simulink model "DPWMA_17_Level_Rectifier_Dual_PI"  (R2021b)
settings: Solver=VariableStepAuto  StartTime=0.0  StopTime=0.5  RelTol=1e-3
libraries: spsSeriesRLCBranchLib x51, spsVoltageMeasurementLib x27, spsDiodeLib x24, spsIGBTDiodeLib x24, simulink x24, spsUniversalBridgeLib x24, slpidlib x3, spsACVoltageSourceLib x3, spsCurrentMeasurementLib x2, spsMeanLib x2, spsRMSLib x2, spsTHDLib x1
(part 3 of 3)

== system DPWMA_17_Level_Rectifier_Dual_PI/Subsystem2/子模块6 ==
  M : Inport
  C : spsSeriesRLCBranchLib/Series RLC Branch  LConnTagsString=__new0  RConnTagsString=__new0  BranchType=C  Resistance=0  Inductance=0  SetiL0=off  InitialCurrent=0  Capacitance=4e-3  Setx0=on  InitialVoltage=1000  Measurements=None
  Diode : spsDiodeLib/Diode  Ron=0.001  Lon=0  Vf=2  IC=0  UseSnubber=0  Rs=1e6  Cs=2e-9  Measurements=off
  IGBT/Diode : spsIGBTDiodeLib/IGBT//Diode  Ron=1e-3  Rs=1e5  Cs=inf  Measurements=off
  R : spsSeriesRLCBranchLib/Series RLC Branch  LConnTagsString=__new0  RConnTagsString=__new0  BranchType=R  Resistance=15  Inductance=0  SetiL0=off  InitialCurrent=0  Capacitance=2e-3  Setx0=on  InitialVoltage=311  Measurements=None
  Subsystem2 : Subsystem
  Universal Bridge : spsUniversalBridgeLib/Universal Bridge  Arms=2  SnubberResistance=0.01  SnubberCapacitance=1e-8  Device=Diodes  Ron=1e-3  Lon=0  ForwardVoltages="[  0  0  ]"  ForwardVoltage=3  GTOparameters=[ 10e-6 , 20e-6 ]  IGBTparameters=[ 1e-6 , 2e-6 ]  Measurements=None  Measurements_2=None  converterType=Rectifier
  Vm1 : spsVoltageMeasurementLib/Voltage Measurement  PhasorSimulation=off  OutputType=Complex  PSBequivalent=0
  + : PMIOPort  Side=Left
  - : PMIOPort  Port=2  Side=Left
  A : PMIOPort  Port=3  Side=Right
  B : PMIOPort  Port=4  Side=Right
  Out1 : Outport
  wires:
  Subsystem2/1(g1) -> IGBT/Diode/1
  M/1 -> Subsystem2/1(MOD)
  Vm1/1 -> Out1/1
  connections:
  Diode/LConn1 -- Universal Bridge/RConn1 -- IGBT/Diode/LConn1
  B/RConn1 -- Universal Bridge/LConn2
  A/RConn1 -- Universal Bridge/LConn1
  Diode/RConn1 -- C/LConn1 -- R/LConn1 -- Vm1/LConn1
  IGBT/Diode/RConn1 -- C/RConn1 -- R/RConn1 -- Vm1/LConn2 -- Universal Bridge/RConn2

== system DPWMA_17_Level_Rectifier_Dual_PI/Subsystem2/子模块7 ==
  M : Inport
  C : spsSeriesRLCBranchLib/Series RLC Branch  LConnTagsString=__new0  RConnTagsString=__new0  BranchType=C  Resistance=0  Inductance=0  SetiL0=off  InitialCurrent=0  Capacitance=4e-3  Setx0=on  InitialVoltage=1000  Measurements=None
  Diode : spsDiodeLib/Diode  Ron=0.001  Lon=0  Vf=2  IC=0  UseSnubber=0  Rs=1e6  Cs=2e-9  Measurements=off
  IGBT/Diode : spsIGBTDiodeLib/IGBT//Diode  Ron=1e-3  Rs=1e5  Cs=inf  Measurements=off
  R : spsSeriesRLCBranchLib/Series RLC Branch  LConnTagsString=__new0  RConnTagsString=__new0  BranchType=R  Resistance=15  Inductance=0  SetiL0=off  InitialCurrent=0  Capacitance=2e-3  Setx0=on  InitialVoltage=311  Measurements=None
  Subsystem2 : Subsystem
  Universal Bridge : spsUniversalBridgeLib/Universal Bridge  Arms=2  SnubberResistance=0.01  SnubberCapacitance=1e-8  Device=Diodes  Ron=1e-3  Lon=0  ForwardVoltages="[  0  0  ]"  ForwardVoltage=3  GTOparameters=[ 10e-6 , 20e-6 ]  IGBTparameters=[ 1e-6 , 2e-6 ]  Measurements=None  Measurements_2=None  converterType=Rectifier
  Vm1 : spsVoltageMeasurementLib/Voltage Measurement  PhasorSimulation=off  OutputType=Complex  PSBequivalent=0
  + : PMIOPort  Side=Left
  - : PMIOPort  Port=2  Side=Left
  A : PMIOPort  Port=3  Side=Right
  B : PMIOPort  Port=4  Side=Right
  Out1 : Outport
  wires:
  Vm1/1 -> Out1/1
  M/1 -> Subsystem2/1(MOD)
  Subsystem2/1(g1) -> IGBT/Diode/1
  connections:
  Universal Bridge/RConn2 -- Vm1/LConn2 -- R/RConn1 -- C/RConn1 -- IGBT/Diode/RConn1
  Vm1/LConn1 -- R/LConn1 -- C/LConn1 -- Diode/RConn1
  A/RConn1 -- Universal Bridge/LConn1
  B/RConn1 -- Universal Bridge/LConn2
  IGBT/Diode/LConn1 -- Universal Bridge/RConn1 -- Diode/LConn1

== system DPWMA_17_Level_Rectifier_Dual_PI/Subsystem2/子模块8 ==
  M : Inport
  C : spsSeriesRLCBranchLib/Series RLC Branch  LConnTagsString=__new0  RConnTagsString=__new0  BranchType=C  Resistance=0  Inductance=0  SetiL0=off  InitialCurrent=0  Capacitance=4e-3  Setx0=on  InitialVoltage=1000  Measurements=None
  Diode : spsDiodeLib/Diode  Ron=0.001  Lon=0  Vf=2  IC=0  UseSnubber=0  Rs=1e6  Cs=2e-9  Measurements=off
  IGBT/Diode : spsIGBTDiodeLib/IGBT//Diode  Ron=1e-3  Rs=1e5  Cs=inf  Measurements=off
  R : spsSeriesRLCBranchLib/Series RLC Branch  LConnTagsString=__new0  RConnTagsString=__new0  BranchType=R  Resistance=15  Inductance=0  SetiL0=off  InitialCurrent=0  Capacitance=2e-3  Setx0=on  InitialVoltage=311  Measurements=None
  Subsystem2 : Subsystem
  Universal Bridge : spsUniversalBridgeLib/Universal Bridge  Arms=2  SnubberResistance=0.01  SnubberCapacitance=1e-8  Device=Diodes  Ron=1e-3  Lon=0  ForwardVoltages="[  0  0  ]"  ForwardVoltage=3  GTOparameters=[ 10e-6 , 20e-6 ]  IGBTparameters=[ 1e-6 , 2e-6 ]  Measurements=None  Measurements_2=None  converterType=Rectifier
  Vm1 : spsVoltageMeasurementLib/Voltage Measurement  PhasorSimulation=off  OutputType=Complex  PSBequivalent=0
  + : PMIOPort  Side=Left
  - : PMIOPort  Port=2  Side=Left
  A : PMIOPort  Port=3  Side=Right
  B : PMIOPort  Port=4  Side=Right
  Out1 : Outport
  wires:
  Subsystem2/1(g1) -> IGBT/Diode/1
  M/1 -> Subsystem2/1(MOD)
  Vm1/1 -> Out1/1
  connections:
  Diode/LConn1 -- Universal Bridge/RConn1 -- IGBT/Diode/LConn1
  B/RConn1 -- Universal Bridge/LConn2
  A/RConn1 -- Universal Bridge/LConn1
  Diode/RConn1 -- C/LConn1 -- R/LConn1 -- Vm1/LConn1
  IGBT/Diode/RConn1 -- C/RConn1 -- R/RConn1 -- Vm1/LConn2 -- Universal Bridge/RConn2

== system DPWMA_17_Level_Rectifier_Dual_PI/Subsystem3/QuTrans ==
  ac : Inport
  Demux : Demux  Outputs=2
  Mux : Mux  Inputs=3
  Sum6 : Sum  Inputs=-|-
  abc : Outport
  wires:
  ac/1 -> Demux/1
  Sum6/1 -> Mux/2
  Demux/1 -> Sum6/1, Mux/1
  Demux/2 -> Sum6/2, Mux/3
  Mux/1 -> abc/1

== system DPWMA_17_Level_Rectifier_Dual_PI/Subsystem3/QuTrans1 ==
  ac : Inport
  Demux : Demux  Outputs=2
  Mux : Mux  Inputs=3
  Sum6 : Sum  Inputs=-|-
  abc : Outport
  wires:
  Mux/1 -> abc/1
  Demux/2 -> Mux/3, Sum6/2
  Demux/1 -> Mux/1, Sum6/1
  Sum6/1 -> Mux/2
  ac/1 -> Demux/1

== system DPWMA_17_Level_Rectifier_Dual_PI/Subsystem/子模块1/Subsystem2 ==
  MOD : Inport
  Abs : Abs
  Relational Operator : RelationalOperator  Operator=<=  OutDataTypeStr=boolean  RndMeth=Nearest
  Triangle1 : simulink/Sources/Repeating Sequence  rep_seq_t=[0 1/2000/2 1/2000]  rep_seq_y=[0 1 0]
  g1 : Outport
  wires:
  MOD/1 -> Abs/1
  Abs/1 -> Relational Operator/1
  Triangle1/1 -> Relational Operator/2
  Relational Operator/1 -> g1/1

== system DPWMA_17_Level_Rectifier_Dual_PI/Subsystem/子模块2/Subsystem2 ==
  MOD : Inport
  Abs : Abs
  Relational Operator : RelationalOperator  Operator=<=  OutDataTypeStr=boolean  RndMeth=Nearest
  Transport Delay : TransportDelay  DelayTime=1/2000/8
  Triangle1 : simulink/Sources/Repeating Sequence  rep_seq_t=[0 1/2000/2 1/2000]  rep_seq_y=[0 1 0]
  g1 : Outport
  wires:
  MOD/1 -> Abs/1
  Triangle1/1 -> Transport Delay/1
  Abs/1 -> Relational Operator/1
  Transport Delay/1 -> Relational Operator/2
  Relational Operator/1 -> g1/1

== system DPWMA_17_Level_Rectifier_Dual_PI/Subsystem/子模块3/Subsystem2 ==
  MOD : Inport
  Abs : Abs
  Relational Operator : RelationalOperator  Operator=<=  OutDataTypeStr=boolean  RndMeth=Nearest
  Transport Delay : TransportDelay  DelayTime=2/2000/8
  Triangle1 : simulink/Sources/Repeating Sequence  rep_seq_t=[0 1/2000/2 1/2000]  rep_seq_y=[0 1 0]
  g1 : Outport
  wires:
  Relational Operator/1 -> g1/1
  Transport Delay/1 -> Relational Operator/2
  Abs/1 -> Relational Operator/1
  Triangle1/1 -> Transport Delay/1
  MOD/1 -> Abs/1

== system DPWMA_17_Level_Rectifier_Dual_PI/Subsystem/子模块4/Subsystem2 ==
  MOD : Inport
  Abs : Abs
  Relational Operator : RelationalOperator  Operator=<=  OutDataTypeStr=boolean  RndMeth=Nearest
  Transport Delay : TransportDelay  DelayTime=3/2000/8
  Triangle1 : simulink/Sources/Repeating Sequence  rep_seq_t=[0 1/2000/2 1/2000]  rep_seq_y=[0 1 0]
  g1 : Outport
  wires:
  MOD/1 -> Abs/1
  Triangle1/1 -> Transport Delay/1
  Abs/1 -> Relational Operator/1
  Transport Delay/1 -> Relational Operator/2
  Relational Operator/1 -> g1/1

== system DPWMA_17_Level_Rectifier_Dual_PI/Subsystem/子模块5/Subsystem2 ==
  MOD : Inport
  Abs : Abs
  Relational Operator : RelationalOperator  Operator=<=  OutDataTypeStr=boolean  RndMeth=Nearest
  Transport Delay : TransportDelay  DelayTime=4/2000/8
  Triangle1 : simulink/Sources/Repeating Sequence  rep_seq_t=[0 1/2000/2 1/2000]  rep_seq_y=[0 1 0]
  g1 : Outport
  wires:
  Relational Operator/1 -> g1/1
  Abs/1 -> Relational Operator/1
  MOD/1 -> Abs/1
  Triangle1/1 -> Transport Delay/1
  Transport Delay/1 -> Relational Operator/2

== system DPWMA_17_Level_Rectifier_Dual_PI/Subsystem/子模块6/Subsystem2 ==
  MOD : Inport
  Abs : Abs
  Relational Operator : RelationalOperator  Operator=<=  OutDataTypeStr=boolean  RndMeth=Nearest
  Transport Delay : TransportDelay  DelayTime=5/2000/8
  Triangle1 : simulink/Sources/Repeating Sequence  rep_seq_t=[0 1/2000/2 1/2000]  rep_seq_y=[0 1 0]
  g1 : Outport
  wires:
  Relational Operator/1 -> g1/1
  Transport Delay/1 -> Relational Operator/2
  Abs/1 -> Relational Operator/1
  Triangle1/1 -> Transport Delay/1
  MOD/1 -> Abs/1

== system DPWMA_17_Level_Rectifier_Dual_PI/Subsystem/子模块7/Subsystem2 ==
  MOD : Inport
  Abs : Abs
  Relational Operator : RelationalOperator  Operator=<=  OutDataTypeStr=boolean  RndMeth=Nearest
  Transport Delay : TransportDelay  DelayTime=6/2000/8
  Triangle1 : simulink/Sources/Repeating Sequence  rep_seq_t=[0 1/2000/2 1/2000]  rep_seq_y=[0 1 0]
  g1 : Outport
  wires:
  MOD/1 -> Abs/1
  Triangle1/1 -> Transport Delay/1
  Abs/1 -> Relational Operator/1
  Transport Delay/1 -> Relational Operator/2
  Relational Operator/1 -> g1/1

== system DPWMA_17_Level_Rectifier_Dual_PI/Subsystem/子模块8/Subsystem2 ==
  MOD : Inport
  Abs : Abs
  Relational Operator : RelationalOperator  Operator=<=  OutDataTypeStr=boolean  RndMeth=Nearest
  Transport Delay : TransportDelay  DelayTime=7/2000/8
  Triangle1 : simulink/Sources/Repeating Sequence  rep_seq_t=[0 1/2000/2 1/2000]  rep_seq_y=[0 1 0]
  g1 : Outport
  wires:
  Relational Operator/1 -> g1/1
  Transport Delay/1 -> Relational Operator/2
  Abs/1 -> Relational Operator/1
  Triangle1/1 -> Transport Delay/1
  MOD/1 -> Abs/1

== system DPWMA_17_Level_Rectifier_Dual_PI/Subsystem1/子模块1/Subsystem2 ==
  MOD : Inport
  Abs : Abs
  Relational Operator : RelationalOperator  Operator=<=  OutDataTypeStr=boolean  RndMeth=Nearest
  Triangle1 : simulink/Sources/Repeating Sequence  rep_seq_t=[0 1/2000/2 1/2000]  rep_seq_y=[0 1 0]
  g1 : Outport
  wires:
  Relational Operator/1 -> g1/1
  Triangle1/1 -> Relational Operator/2
  Abs/1 -> Relational Operator/1
  MOD/1 -> Abs/1

== system DPWMA_17_Level_Rectifier_Dual_PI/Subsystem1/子模块2/Subsystem2 ==
  MOD : Inport
  Abs : Abs
  Relational Operator : RelationalOperator  Operator=<=  OutDataTypeStr=boolean  RndMeth=Nearest
  Transport Delay : TransportDelay  DelayTime=1/2000/8
  Triangle1 : simulink/Sources/Repeating Sequence  rep_seq_t=[0 1/2000/2 1/2000]  rep_seq_y=[0 1 0]
  g1 : Outport
  wires:
  Relational Operator/1 -> g1/1
  Transport Delay/1 -> Relational Operator/2
  Abs/1 -> Relational Operator/1
  Triangle1/1 -> Transport Delay/1
  MOD/1 -> Abs/1

== system DPWMA_17_Level_Rectifier_Dual_PI/Subsystem1/子模块3/Subsystem2 ==
  MOD : Inport
  Abs : Abs
  Relational Operator : RelationalOperator  Operator=<=  OutDataTypeStr=boolean  RndMeth=Nearest
  Transport Delay : TransportDelay  DelayTime=2/2000/8
  Triangle1 : simulink/Sources/Repeating Sequence  rep_seq_t=[0 1/2000/2 1/2000]  rep_seq_y=[0 1 0]
  g1 : Outport
  wires:
  MOD/1 -> Abs/1
  Triangle1/1 -> Transport Delay/1
  Abs/1 -> Relational Operator/1
  Transport Delay/1 -> Relational Operator/2
  Relational Operator/1 -> g1/1

== system DPWMA_17_Level_Rectifier_Dual_PI/Subsystem1/子模块4/Subsystem2 ==
  MOD : Inport
  Abs : Abs
  Relational Operator : RelationalOperator  Operator=<=  OutDataTypeStr=boolean  RndMeth=Nearest
  Transport Delay : TransportDelay  DelayTime=3/2000/8
  Triangle1 : simulink/Sources/Repeating Sequence  rep_seq_t=[0 1/2000/2 1/2000]  rep_seq_y=[0 1 0]
  g1 : Outport
  wires:
  Relational Operator/1 -> g1/1
  Transport Delay/1 -> Relational Operator/2
  Abs/1 -> Relational Operator/1
  Triangle1/1 -> Transport Delay/1
  MOD/1 -> Abs/1

== system DPWMA_17_Level_Rectifier_Dual_PI/Subsystem1/子模块5/Subsystem2 ==
  MOD : Inport
  Abs : Abs
  Relational Operator : RelationalOperator  Operator=<=  OutDataTypeStr=boolean  RndMeth=Nearest
  Transport Delay : TransportDelay  DelayTime=4/2000/8
  Triangle1 : simulink/Sources/Repeating Sequence  rep_seq_t=[0 1/2000/2 1/2000]  rep_seq_y=[0 1 0]
  g1 : Outport
  wires:
  Transport Delay/1 -> Relational Operator/2
  Triangle1/1 -> Transport Delay/1
  MOD/1 -> Abs/1
  Abs/1 -> Relational Operator/1
  Relational Operator/1 -> g1/1

== system DPWMA_17_Level_Rectifier_Dual_PI/Subsystem1/子模块6/Subsystem2 ==
  MOD : Inport
  Abs : Abs
  Relational Operator : RelationalOperator  Operator=<=  OutDataTypeStr=boolean  RndMeth=Nearest
  Transport Delay : TransportDelay  DelayTime=5/2000/8
  Triangle1 : simulink/Sources/Repeating Sequence  rep_seq_t=[0 1/2000/2 1/2000]  rep_seq_y=[0 1 0]
  g1 : Outport
  wires:
  MOD/1 -> Abs/1
  Triangle1/1 -> Transport Delay/1
  Abs/1 -> Relational Operator/1
  Transport Delay/1 -> Relational Operator/2
  Relational Operator/1 -> g1/1

== system DPWMA_17_Level_Rectifier_Dual_PI/Subsystem1/子模块7/Subsystem2 ==
  MOD : Inport
  Abs : Abs
  Relational Operator : RelationalOperator  Operator=<=  OutDataTypeStr=boolean  RndMeth=Nearest
  Transport Delay : TransportDelay  DelayTime=6/2000/8
  Triangle1 : simulink/Sources/Repeating Sequence  rep_seq_t=[0 1/2000/2 1/2000]  rep_seq_y=[0 1 0]
  g1 : Outport
  wires:
  Relational Operator/1 -> g1/1
  Transport Delay/1 -> Relational Operator/2
  Abs/1 -> Relational Operator/1
  Triangle1/1 -> Transport Delay/1
  MOD/1 -> Abs/1

== system DPWMA_17_Level_Rectifier_Dual_PI/Subsystem1/子模块8/Subsystem2 ==
  MOD : Inport
  Abs : Abs
  Relational Operator : RelationalOperator  Operator=<=  OutDataTypeStr=boolean  RndMeth=Nearest
  Transport Delay : TransportDelay  DelayTime=7/2000/8
  Triangle1 : simulink/Sources/Repeating Sequence  rep_seq_t=[0 1/2000/2 1/2000]  rep_seq_y=[0 1 0]
  g1 : Outport
  wires:
  MOD/1 -> Abs/1
  Triangle1/1 -> Transport Delay/1
  Abs/1 -> Relational Operator/1
  Transport Delay/1 -> Relational Operator/2
  Relational Operator/1 -> g1/1

== system DPWMA_17_Level_Rectifier_Dual_PI/Subsystem2/子模块1/Subsystem2 ==
  MOD : Inport
  Abs : Abs
  Relational Operator : RelationalOperator  Operator=<=  OutDataTypeStr=boolean  RndMeth=Nearest
  Triangle1 : simulink/Sources/Repeating Sequence  rep_seq_t=[0 1/2000/2 1/2000]  rep_seq_y=[0 1 0]
  g1 : Outport
  wires:
  MOD/1 -> Abs/1
  Abs/1 -> Relational Operator/1
  Triangle1/1 -> Relational Operator/2
  Relational Operator/1 -> g1/1

== system DPWMA_17_Level_Rectifier_Dual_PI/Subsystem2/子模块2/Subsystem2 ==
  MOD : Inport
  Abs : Abs
  Relational Operator : RelationalOperator  Operator=<=  OutDataTypeStr=boolean  RndMeth=Nearest
  Transport Delay : TransportDelay  DelayTime=1/2000/8
  Triangle1 : simulink/Sources/Repeating Sequence  rep_seq_t=[0 1/2000/2 1/2000]  rep_seq_y=[0 1 0]
  g1 : Outport
  wires:
  MOD/1 -> Abs/1
  Triangle1/1 -> Transport Delay/1
  Abs/1 -> Relational Operator/1
  Transport Delay/1 -> Relational Operator/2
  Relational Operator/1 -> g1/1

== system DPWMA_17_Level_Rectifier_Dual_PI/Subsystem2/子模块3/Subsystem2 ==
  MOD : Inport
  Abs : Abs
  Relational Operator : RelationalOperator  Operator=<=  OutDataTypeStr=boolean  RndMeth=Nearest
  Transport Delay : TransportDelay  DelayTime=2/2000/8
  Triangle1 : simulink/Sources/Repeating Sequence  rep_seq_t=[0 1/2000/2 1/2000]  rep_seq_y=[0 1 0]
  g1 : Outport
  wires:
  Relational Operator/1 -> g1/1
  Transport Delay/1 -> Relational Operator/2
  Abs/1 -> Relational Operator/1
  Triangle1/1 -> Transport Delay/1
  MOD/1 -> Abs/1

== system DPWMA_17_Level_Rectifier_Dual_PI/Subsystem2/子模块4/Subsystem2 ==
  MOD : Inport
  Abs : Abs
  Relational Operator : RelationalOperator  Operator=<=  OutDataTypeStr=boolean  RndMeth=Nearest
  Transport Delay : TransportDelay  DelayTime=3/2000/8
  Triangle1 : simulink/Sources/Repeating Sequence  rep_seq_t=[0 1/2000/2 1/2000]  rep_seq_y=[0 1 0]
  g1 : Outport
  wires:
  MOD/1 -> Abs/1
  Triangle1/1 -> Transport Delay/1
  Abs/1 -> Relational Operator/1
  Transport Delay/1 -> Relational Operator/2
  Relational Operator/1 -> g1/1

== system DPWMA_17_Level_Rectifier_Dual_PI/Subsystem2/子模块5/Subsystem2 ==
  MOD : Inport
  Abs : Abs
  Relational Operator : RelationalOperator  Operator=<=  OutDataTypeStr=boolean  RndMeth=Nearest
  Transport Delay : TransportDelay  DelayTime=4/2000/8
  Triangle1 : simulink/Sources/Repeating Sequence  rep_seq_t=[0 1/2000/2 1/2000]  rep_seq_y=[0 1 0]
  g1 : Outport
  wires:
  Relational Operator/1 -> g1/1
  Abs/1 -> Relational Operator/1
  MOD/1 -> Abs/1
  Triangle1/1 -> Transport Delay/1
  Transport Delay/1 -> Relational Operator/2

== system DPWMA_17_Level_Rectifier_Dual_PI/Subsystem2/子模块6/Subsystem2 ==
  MOD : Inport
  Abs : Abs
  Relational Operator : RelationalOperator  Operator=<=  OutDataTypeStr=boolean  RndMeth=Nearest
  Transport Delay : TransportDelay  DelayTime=5/2000/8
  Triangle1 : simulink/Sources/Repeating Sequence  rep_seq_t=[0 1/2000/2 1/2000]  rep_seq_y=[0 1 0]
  g1 : Outport
  wires:
  Relational Operator/1 -> g1/1
  Transport Delay/1 -> Relational Operator/2
  Abs/1 -> Relational Operator/1
  Triangle1/1 -> Transport Delay/1
  MOD/1 -> Abs/1

== system DPWMA_17_Level_Rectifier_Dual_PI/Subsystem2/子模块7/Subsystem2 ==
  MOD : Inport
  Abs : Abs
  Relational Operator : RelationalOperator  Operator=<=  OutDataTypeStr=boolean  RndMeth=Nearest
  Transport Delay : TransportDelay  DelayTime=6/2000/8
  Triangle1 : simulink/Sources/Repeating Sequence  rep_seq_t=[0 1/2000/2 1/2000]  rep_seq_y=[0 1 0]
  g1 : Outport
  wires:
  MOD/1 -> Abs/1
  Triangle1/1 -> Transport Delay/1
  Abs/1 -> Relational Operator/1
  Transport Delay/1 -> Relational Operator/2
  Relational Operator/1 -> g1/1

== system DPWMA_17_Level_Rectifier_Dual_PI/Subsystem2/子模块8/Subsystem2 ==
  MOD : Inport
  Abs : Abs
  Relational Operator : RelationalOperator  Operator=<=  OutDataTypeStr=boolean  RndMeth=Nearest
  Transport Delay : TransportDelay  DelayTime=7/2000/8
  Triangle1 : simulink/Sources/Repeating Sequence  rep_seq_t=[0 1/2000/2 1/2000]  rep_seq_y=[0 1 0]
  g1 : Outport
  wires:
  Relational Operator/1 -> g1/1
  Transport Delay/1 -> Relational Operator/2
  Abs/1 -> Relational Operator/1
  Triangle1/1 -> Transport Delay/1
  MOD/1 -> Abs/1
